simulink library "Spring_Control_Axle3"  (R2025a)
settings: Solver=VariableStepAuto  StartTime=0.0  StopTime=10.0  RelTol=1e-3
libraries: Spring_Control x3, Vehicle_Outputs x1
Description:
  | Copyright 2026 The MathWorks, Inc.
settings Model: Creator=smiller  LastModifiedBy=smiller
settings OptimizationCC: ReuseModelBlockBuffer=off
settings ModelReferenceCC: EnableRefExpFcnMdlSchedulingChecks=on
settings RTWCC: GPUComputeCapability=3.5

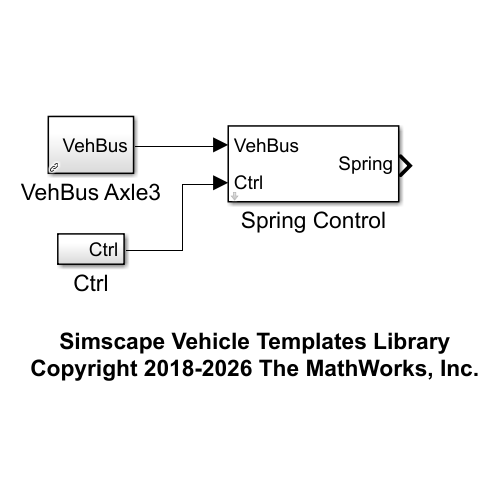
[thumbnail: Simulink's stored preview of the top-level diagram]
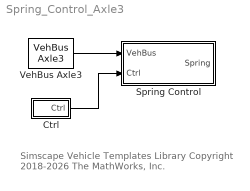
== system Spring_Control_Axle3 ==
  note: Simscape Vehicle Templates Library
      | Copyright 2018-2026 The MathWorks, Inc.
  Ctrl : Subsystem
  Spring Control : Subsystem  mask(Spring Control, Three Axle){popup_spring_control_A1=None, popup_spring_control_A2=None, popup_spring_control_A3=None}
      mask prompts: popup_spring_control_A1 "Spring Control Axle 1"; popup_spring_control_A2 "Spring Control Axle 2"; popup_spring_control_A3 "Spring Control Axle 3"
      mask help: Configurable spring control for three axles, left and right sides.
      mask TypeOptions popup_spring_control_A1: Spring Control A1/popup_spring_control
      mask TypeOptions popup_spring_control_A2: Spring Control A2/popup_spring_control
      mask TypeOptions popup_spring_control_A3: Spring Control A3/popup_spring_control
  VehBus Axle3 : Vehicle_Outputs/VehBus Axle3  SystemSampleTime=-1  VariantActivationTime=update diagram  EmptyChoice=off  PassThrough=off  PassThroughVariantControl=(default)  EmptyChoiceVariantControl=(default)  AllowFlexibleInterface=on  Latency=0  AutoFrameSizeCalculation=off
  wires:
  VehBus Axle3/1 -> Spring Control/1(VehBus)
  Ctrl/1(Ctrl) -> Spring Control/2(Ctrl)

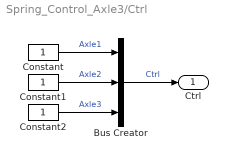
== system Spring_Control_Axle3/Ctrl ==
  Bus Creator : BusCreator  Inputs=3
  Constant : Constant
  Constant1 : Constant
  Constant2 : Constant
  Ctrl : Outport
  wires:
  Constant/1 -> Bus Creator/1  "Axle1"
  Constant1/1 -> Bus Creator/2  "Axle2"
  Bus Creator/1 -> Ctrl/1  "Ctrl"
  Constant2/1 -> Bus Creator/3  "Axle3"

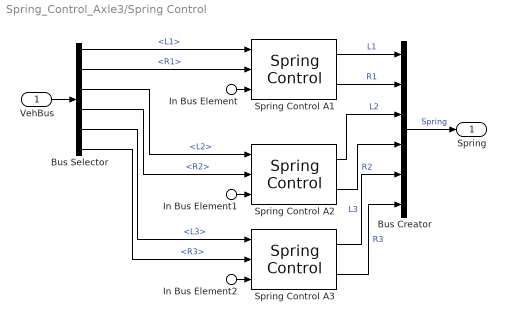
== system Spring_Control_Axle3/Spring Control ==
  VehBus : Inport
  In Bus Element : Inport  Port=2  PortName=Ctrl  Element=Axle1
  In Bus Element1 : Inport  Port=2  PortName=Ctrl  Element=Axle2
  In Bus Element2 : Inport  Port=2  PortName=Ctrl  Element=Axle3
  Bus Creator : BusCreator  Inputs=6
  Bus Selector : BusSelector  OutputSignals=Chassis.Spring.L1,Chassis.Spring.R1,Chassis.Spring.L2,Chassis.Spring.R2,Chassis.Spring.L3,Chassis.Spring.R3
  Spring Control A1 : Spring_Control/Spring Control  VariantControl=Choice  LabelModeActiveChoice=None  popup_spring_control=None  popup_gas_spring=Stiff
  Spring Control A2 : Spring_Control/Spring Control  VariantControl=Choice  LabelModeActiveChoice=None  popup_spring_control=None  popup_gas_spring=Stiff
  Spring Control A3 : Spring_Control/Spring Control  VariantControl=Choice  LabelModeActiveChoice=None  popup_spring_control=None  popup_gas_spring=Stiff
  Spring : Outport
  wires:
  VehBus/1 -> Bus Selector/1
  Spring Control A1/1 -> Bus Creator/1  "L1"
  Bus Selector/1 -> Spring Control A1/1  "<L1>"
  Bus Selector/2 -> Spring Control A1/2  "<R1>"
  Bus Selector/3 -> Spring Control A2/1  "<L2>"
  Bus Selector/4 -> Spring Control A2/2  "<R2>"
  Bus Creator/1 -> Spring/1  "Spring"
  Spring Control A1/2 -> Bus Creator/2  "R1"
  Spring Control A2/1 -> Bus Creator/3  "L2"
  Spring Control A2/2 -> Bus Creator/4  "R2"
  In Bus Element/1 -> Spring Control A1/3
  In Bus Element1/1 -> Spring Control A2/3
  Bus Selector/5 -> Spring Control A3/1  "<L3>"
  Bus Selector/6 -> Spring Control A3/2  "<R3>"
  Spring Control A3/1 -> Bus Creator/5  "L3"
  Spring Control A3/2 -> Bus Creator/6  "R3"
  In Bus Element2/1 -> Spring Control A3/3
